simulink model "StateflowChart"  (R2026a)
settings: Solver=VariableStepAuto  StopTime=60
StartFcn:
  | learning.simulink.modelCallbacks.startFunction(gcs);
StopFcn:
  | learning.simulink.modelCallbacks.stopFunction(gcs);
model workspace (MAT data in the model file):
  courseObject.course = 'stateflow'
  courseObject.chapter = 2
  courseObject.lesson = 2
  courseObject.section = 1
  courseObject.task = 1
  t_ans = [0; 1; 2; 3; 4; 5; 6; 7; 8; 9; 10; 11; 12; 13; 14; 15; 16; 17; 18; 19; 20; 21; 22; 23; 24; 25; 26; 27; 28; 29; 30; 31; 32; 33; 34; 35; 36; 37; 38; 39; 40; 41; 42; 43; 44; 45; 46; 47; 48; 49; 50; 51; 52; 53; 54; 55; 56; 57; 58; 59; 60]
  y_ans = [1; 1; 1; 0; 0; 0; 0; 0; 0; 0; 0; 0; 0; 0; 1; 0; 1; 0; 1; 0; 1; 1; 1; 0; 0; 0; 0; 0; 0; 0; 1; 0; 1; 0; 1; 0; 1; 0; 1; 1; 1; 0; 0; 0; 0; 0; 0; 0; 0; 0; 0; 0; 0; 0; 0; 0; 0; 0; 0; 1; 1]
libraries: signalChecks x1, SignalEditorBlockLib x1
CloseFcn:
  | learning.simulink.cleanupOnlineTraining;learning.simulink.Application.getInstance().dduxLogMatlabEvent("ModelClosed");
Description:
  | TrainingCourseModel
settings Model: Creator=PC  LastModifiedBy=PC

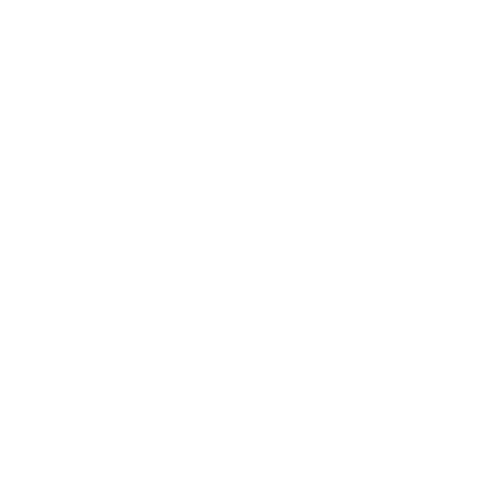
[thumbnail: Simulink's stored preview of the top-level diagram]
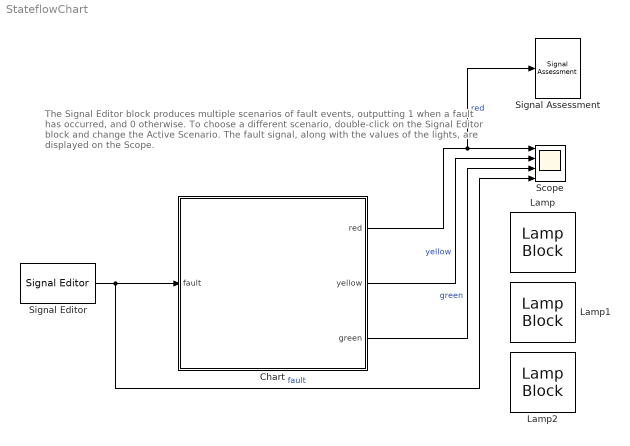
== system StateflowChart ==
  note: The Signal Editor block produces multiple scenarios of fault events, outputting 1 when a fault has occurred, and 0 otherwise.
      |
      | To choose a different scenario, double-click on the Signal Editor block and change the Active Scenario.
      |
      | The fault signal, along with the values of the lights, are displayed on the Scope.
  Chart : Stateflow chart  TreatAsAtomicUnit=on
  Lamp : LampBlock  LabelPosition=Hide  DefaultColor=[192.0, 192.0, 192.0]
  Lamp1 : LampBlock  LabelPosition=Hide  DefaultColor=[192.0, 192.0, 192.0]
  Lamp2 : LampBlock  LabelPosition=Hide  DefaultColor=[192.0, 192.0, 192.0]
  Scope : Scope  NumInputPorts=4
      settings: ActiveDisplayYMinimum=-0.125  ActiveDisplayYMaximum=1.125
  Signal Assessment : signalChecks/Signal Assessment  signal_type='signal'  t_ans=t_ans  y_ans_upper=y_ans  y_ans_lower=0  range=0.005  rate_type=1  lesson=0  task=4  pass=1
  Signal Editor : SignalEditorBlockLib/Signal Editor  FileName=trafficLightFault.mat  ActiveScenario=Faults  ActiveSignal=fault  IsBus=off  OutputBusObjectStr=Bus: BusObject  SampleTime=1  Interpolate=off  ZeroCross=off  OutputAfterFinalValue=Setting to zero  Unit=inherit  PreserveSignalName=on  ApplySigPropsToAllScenarios=on  ApplySigPropsToAllSignals=off  SignalPropertySource=Dialog parameters
  wires:
  Chart/3(green) -> Scope/3  "green"
  Signal Editor/1 -> Chart/1(fault), Scope/4  "fault"
  Chart/1(red) -> Signal Assessment/1, Scope/1  "red"
  Chart/2(yellow) -> Scope/2  "yellow"

== stateflow chart StateflowChart/Chart ==
  note: In this chart, entering a state sets the individual lamps (red, yellow, and green) to either on ( 1 ) or off ( 0 ).
      |
      | There are two operating modes.
      | Normal: The traffic light rotates between red, yellow, and green based on a timer.
      | Fault: The traffic light turns the red lamp off and on based on a timer.
  state Normal
    state Stop
      % Red light
      entry:
      red = 1;
      yellow = 0;
      green = 0;
    state PrepareToStop
      % Yellow light
      entry:
      red = 0;
      yellow = 1;
      green = 0;
    state Go
      % Green light
      entry:
      red = 0;
      yellow = 0;
      green = 1;
    (default) -> Stop
    Stop -> (junction 26)
    (junction 26) -> (junction 29) : after(3,sec)
    PrepareToStop -> Stop : after(3,sec)
    Go -> PrepareToStop : after(15,sec)
    (junction 29) -> Go
  state Fault
    entry:
    yellow = 0;
    green = 0;
    state BlinkOn
      % Red light
      entry:
      red = 1;
    state BlinkOff
      % No light
      entry:
      red = 0;
    (default) -> BlinkOn
    BlinkOff -> BlinkOn : after(1,sec)
    BlinkOn -> BlinkOff : after(1,sec)
  (default) -> Normal
  Normal -> Fault : [fault == 1]
  Fault -> Normal : [fault == 0]
  data: red output =1; yellow output; fault input; green output =0
